simulink model "FS_PWT_Control_and_Motor"  (R2025b)
settings: Solver=FixedStepAuto  StartTime=0.0  StopTime=17  FixedStep=2e-5  RelTol=1e-3
values from neighbouring files (symbols this model uses):
  B_m = 1e-4    (= 0.0001)    [Example_parameters.m]
  Fm = 0.028    [Example_parameters.m]
  J_eq = J_m + 0.032    (= 0.032274)    [Example_parameters.m]
  Ld = 0.12e-3    (= 0.00012)    [Example_parameters.m]
  Lq = 0.24e-3    (= 0.00024)    [Example_parameters.m]
  n_max = 20000    [Example_parameters.m]
  nm_ref = n_max    (= 20000)    [Example_parameters.m]
  p = 5    [Example_parameters.m]
  R_s = 0.135    [Example_parameters.m]
  t0 = 0.2    [Example_parameters.m]
  T1 = 0.9*T_max    (= 18)    [Example_parameters.m]
  t1 = t0+5    (= 5.2)    [Example_parameters.m]
  T2 = -T_rated    (= -9.8)    [Example_parameters.m]
  t2 = t1+10    (= 15.2)    [Example_parameters.m]
  Torque_set_matrix = [379.08 379.13 379.18 379.23 379.28 379.33 379.38 379.43 379.48 379.53 379.58 379.63 ... (678 elements, 339x2)]    [Example_torque_reference.mat]
  V_dc = 600    [Example_parameters.m]
libraries: eeTransforms x3
settings Model: SimulationMode=accelerator  Creator=giuli  LastModifiedBy=giuli

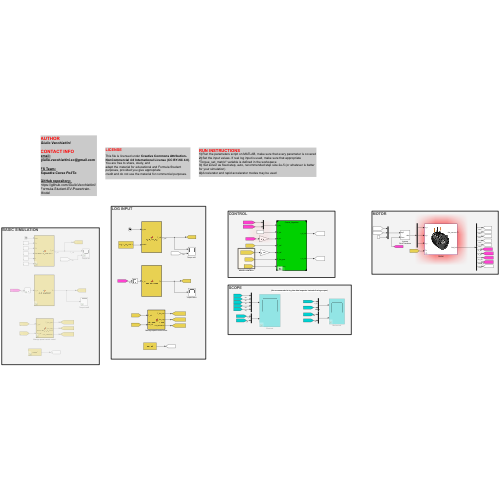
[thumbnail: Simulink's stored preview of the top-level diagram]
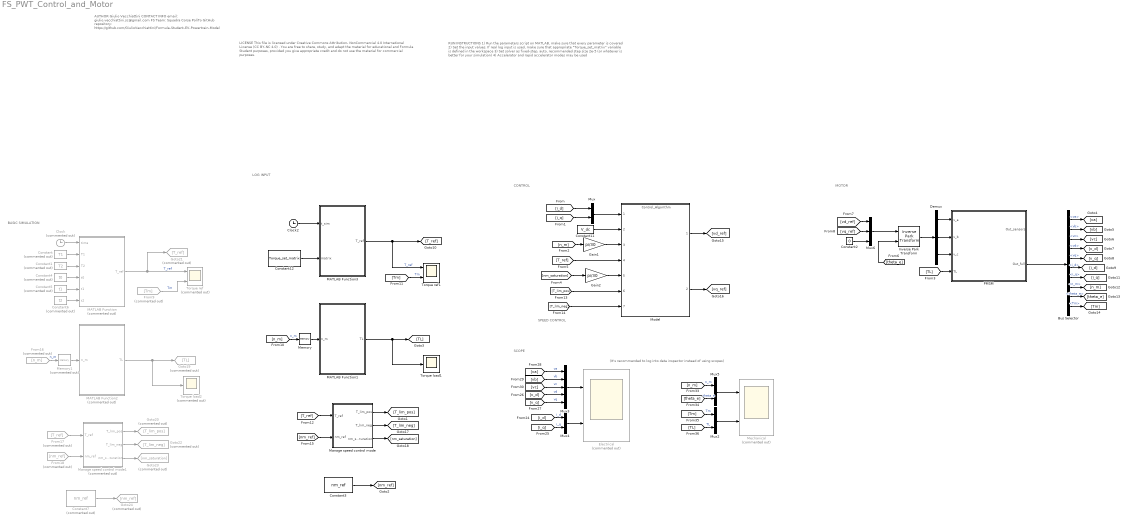
== system FS_PWT_Control_and_Motor ==
  note: (It's recommended to log into data inspector instead of using scopes)
  note: BASIC SIMULATION
  note: LOG INPUT
  note: SCOPE
  note: SPEED CONTROL
  note: CONTROL
  note: MOTOR
  note: LICENSE
      |
      | This file is licensed under Creative Commons Attribution-
      | NonCommercial 4.0 International License (CC BY-NC 4.0) . You are free to share, study, and
      | adapt the material for educational and Formula Student purposes, provided you give appropriate
      | credit and do not use the material for commercial purposes.
  note: RUN INSTRUCTIONS
      | 1) Run the parameters script on MATLAB, make sure that every parameter is covered
      | 2) Set the input values. If real log input is used, make sure that appropriate "Torque_set_matrix" variable is defined in the workspace
      | 3) Set solver as fixed-step, auto, recommended step size 2e-5 (or whatever is better for your simulation)
      | 4) Accelerator and rapid accelerator modes may be used
  note: AUTHOR
      | Giulio Vecchiattini
      |
      | CONTACT INFO
      | email: giulio.vecchiattini.sc@gmail.com
      |
      | FS Team:
      | Squadra Corse PoliTo
      |
      | GitHub repository:
      | https://github.com/GiulioVecchiattini/Formula-Student-EV-Powertrain-Model
  Bus Selector : BusSelector  OutputSignals=va,vb,vc,vd,vq,i_d,i_q,n_m,theta_e,Tm
  Clock : Clock  Commented=on
  Clock2 : Clock
  Constant : Constant  Commented=on  Value=T1
  Constant1 : Constant  Commented=on  Value=T2
  Constant11 : Constant  Value=V_dc
  Constant12 : Constant  Value=Torque_set_matrix
  Constant2 : Constant  Value=0
  Constant3 : Constant  Value=nm_ref
  Constant4 : Constant  Commented=on  Value=t0
  Constant5 : Constant  Commented=on  Value=t1
  Constant6 : Constant  Commented=on  Value=t2
  Constant7 : Constant  Commented=on  Value=nm_ref
  Demux : Demux  Outputs=3
  Electrical : Scope  Commented=on  NumInputPorts=2
      settings: ActiveDisplayYMinimum=-222.33483903014351  ActiveDisplayYMaximum=248.98362192273623
  From16 : From  Commented=on  GotoTag=n_m
  From17 : From  Commented=on  GotoTag=T_ref
  From18 : From  Commented=on  GotoTag=nm_ref
  From9 : From  Commented=on  GotoTag=Tm
  Gain1 : Gain  Gain=pi/30
  Gain2 : Gain  Gain=pi/30
  Goto19 : Goto  Commented=on  GotoTag=TL
  Goto20 : Goto  Commented=on  GotoTag=T_lim_pos
  Goto21 : Goto  Commented=on  GotoTag=T_ref
  Goto22 : Goto  Commented=on  GotoTag=T_lim_neg
  Goto23 : Goto  Commented=on  GotoTag=nm_saturation
  Goto24 : Goto  Commented=on  GotoTag=nm_ref
  Inverse Park Transform : eeTransforms/Inverse Park Transform  AxisAlignment=D-axis  PowerInvariant=off
      settings: LibrarySourceBlock=|
      | ee_sl_lib/Mathematical
      | Transforms/Inverse
      | Park Transform
  MATLAB Function : MATLAB Function  Commented=on  TreatAsAtomicUnit=on
  MATLAB Function1 : MATLAB Function  TreatAsAtomicUnit=on
  MATLAB Function2 : MATLAB Function  Commented=on  TreatAsAtomicUnit=on
  MATLAB Function3 : MATLAB Function  TreatAsAtomicUnit=on
  Manage speed control mode : MATLAB Function  TreatAsAtomicUnit=on
  Manage speed control mode1 : MATLAB Function  Commented=on  TreatAsAtomicUnit=on
  Mechanical : Scope  Commented=on  NumInputPorts=2
      settings: ActiveDisplayYMinimum=-1910.5368954552505  ActiveDisplayYMaximum=17194.832059097258  DataLoggingVariableName=ScopeData2
  Memory : Memory
  Memory1 : Memory  Commented=on
  Model : ModelReference  ModelNameDialog=Control_Algorithm.slxp  UsingDefaultArgumentValue=0,0,0,0,0,0,0,0,0,0,0,0,0,0,0,0,0,0,0  ModelReferenceVersion=1.7  CopyOfModelProtected=on  Torque_control=1  T_max=T_max  V_dc_max=V_dc_max  V_max=V_max  k_T=k_T  I_max=I_max  Kp_d=Kp_d  Ki_d=Ki_d  Kp_q=Kp_q  Ki_q=Ki_q  Kp_n=Kp_n  Ki_n=Ki_n  Kd_n=Kd_n  Kp_v=Kp_v  Ki_v=Ki_v  n_lim_brake=0.02*n_max  n_min_brake=0.01*n_max  n_max=n_max*1.02  n_lim=0.95*n_max
  Mux{,2,4..5} (4 alike) : Mux  Inputs=2
  Mux3 : Mux  Inputs=5
  Mux6 : Mux  Inputs=3
  PMSM : Subsystem  mask(PMSM){Ld=Ld, Lq=Lq, Fm=Fm, R_s=R_s, p=p, J_eq=J_eq, B_m=B_m}
      mask prompts: Ld "Ld (H)"; Lq "Lq (H)"; Fm "Magnet flux linkage (Vs)"; R_s "Rs (Ohm)"; p "Pole pairs p"; J_eq "Equivalent inertia [kg*m^2]"; B_m "Viscous friction [N*s/m]"
      mask help: Simplified PMSM with constant Ld, Lq, Fm
      mask Display: image('PMSM.jpg');
  Torque load1 : Scope
      settings: ActiveDisplayYMinimum=-1.2249999999999999  ActiveDisplayYMaximum=11.025  DataLoggingVariableName=ScopeData4
  Torque load2 : Scope  Commented=on
      settings: ActiveDisplayYMinimum=-1.2249999999999999  ActiveDisplayYMaximum=11.025
  Torque ref : Scope  Commented=on  NumInputPorts=2
      settings: ActiveDisplayYMinimum=-25.856939038681524  ActiveDisplayYMaximum=25.9527334054476  DataLoggingVariableName=ScopeData3
  Torque ref1 : Scope  NumInputPorts=2
      settings: ActiveDisplayYMinimum=-1.08125401214301  ActiveDisplayYMaximum=9.7312861092870921  DataLoggingVariableName=ScopeData5
  wires:
  Model/1 -> [vd_ref]
  Manage speed control mode/2(T_lim_neg) -> [T_lim_neg]
  [nm_saturation] -> Gain2/1
  Bus Selector/6 -> [i_d]  "<i_d>"
  Mux4/1 -> Electrical/2
  [v_q] -> Mux3/5  "vq"
  Bus Selector/3 -> [vc]  "<vc>"
  Constant5/1 -> MATLAB Function/5(t1)
  Constant11/1 -> Model/2
  [i_q] -> Mux4/2  "i_q"
  Gain2/1 -> Model/5
  Constant6/1 -> MATLAB Function/6(t2)
  MATLAB Function/1(T_ref) -> Goto21/1, Torque ref/1  "T_ref"
  Manage speed control mode/1(T_lim_pos) -> [T_lim_pos]
  From9/1 -> Torque ref/2  "Tm"
  [vd_ref] -> Mux6/1
  [vc] -> Mux3/3  "vc"
  Constant/1 -> MATLAB Function/2(T1)
  Bus Selector/9 -> [theta_e]  "<theta_e>"
  Mux2/1 -> Mechanical/2
  [T_ref] -> Manage speed control mode/1(T_ref)
  Demux/2 -> PMSM/2(v_b)
  Demux/3 -> PMSM/3(v_c)
  Constant12/1 -> MATLAB Function3/2(matrix)
  Bus Selector/10 -> [Tm]  "<Tm>"
  Bus Selector/8 -> [n_m]  "<n_m>"
  Constant3/1 -> [nm_ref]
  Mux6/1 -> Inverse Park Transform/1
  Bus Selector/5 -> [v_q]  "<vq>"
  Clock/1 -> MATLAB Function/1(time)
  [i_d] -> Mux/1
  [TL] -> Mux2/2  "TL"
  [Tm] -> Torque ref1/2  "Tm"
  Inverse Park Transform/1 -> Demux/1
  [T_ref] -> Model/4
  [va] -> Mux3/1  "va"
  MATLAB Function3/1(T_ref) -> [T_ref], Torque ref1/1  "T_ref"
  [n_m] -> Gain1/1
  Manage speed control mode/3(nm_saturation) -> [nm_saturation]
  [TL] -> PMSM/4(TL)
  [theta_e] -> Mux5/2  "theta_e"
  [n_m] -> Memory/1  "n_m"
  Memory/1 -> MATLAB Function1/1(n_m)
  Bus Selector/7 -> [i_q]  "<i_q>"
  [T_lim_neg] -> Model/7
  [Tm] -> Mux2/1  "Tm"
  Constant2/1 -> Mux6/3
  [i_d] -> Mux4/1  "i_d"
  [nm_ref] -> Manage speed control mode/2(nm_ref)
  Constant1/1 -> MATLAB Function/3(T2)
  [theta_e] -> Inverse Park Transform/2
  PMSM/2(Out_full) -> Bus Selector/1
  Constant4/1 -> MATLAB Function/4(t0)
  Bus Selector/4 -> [v_d]  "<vd>"
  Bus Selector/2 -> [vb]  "<vb>"
  Mux5/1 -> Mechanical/1
  [n_m] -> Mux5/1  "n_m"
  Mux3/1 -> Electrical/1
  Clock2/1 -> MATLAB Function3/1(t_sim)
  Mux/1 -> Model/1
  [T_lim_pos] -> Model/6
  Demux/1 -> PMSM/1(v_a)
  Model/2 -> [vq_ref]
  Bus Selector/1 -> [va]  "<va>"
  [v_d] -> Mux3/4  "vd"
  [i_q] -> Mux/2
  [vq_ref] -> Mux6/2
  Gain1/1 -> Model/3
  [vb] -> Mux3/2  "vb"
  MATLAB Function1/1(TL) -> [TL], Torque load1/1
  MATLAB Function2/1(TL) -> Goto19/1, Torque load2/1
  Memory1/1 -> MATLAB Function2/1(n_m)
  From16/1 -> Memory1/1  "n_m"
  From18/1 -> Manage speed control mode1/2(nm_ref)
  Manage speed control mode1/3(nm_saturation) -> Goto23/1
  From17/1 -> Manage speed control mode1/1(T_ref)
  Manage speed control mode1/1(T_lim_pos) -> Goto20/1
  Manage speed control mode1/2(T_lim_neg) -> Goto22/1
  Constant7/1 -> Goto24/1

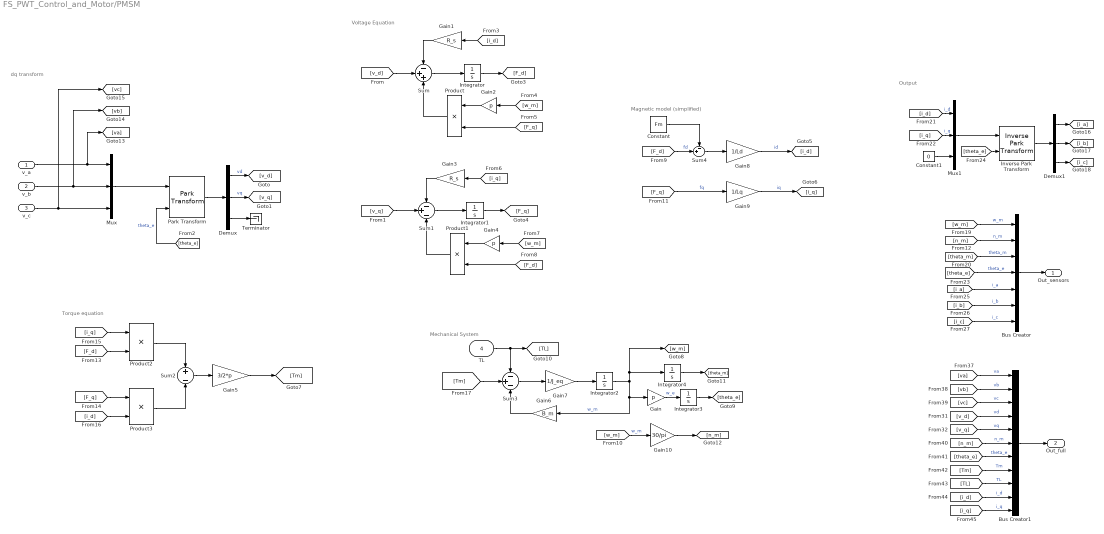
== system FS_PWT_Control_and_Motor/PMSM ==
  note: Output
  note: Magnetic model (simplified)
  note: Mechanical System
  note: Torque equation
  note: dq transform
  note: Voltage Equation
  v_a : Inport
  v_b : Inport  Port=2
  v_c : Inport  Port=3
  TL : Inport  Port=4
  Bus Creator : BusCreator  Inputs=7
  Bus Creator1 : BusCreator  Inputs=11
  Constant : Constant  Value=Fm
  Constant1 : Constant  Value=0
  Demux : Demux  Outputs=3
  Demux1 : Demux  Outputs=3
  Gain : Gain  Gain=p
  Gain1 : Gain  Gain=R_s
  Gain10 : Gain  Gain=30/pi
  Gain2 : Gain  Gain=p
  Gain3 : Gain  Gain=R_s
  Gain4 : Gain  Gain=p
  Gain5 : Gain  Gain=3/2*p
  Gain6 : Gain  Gain=B_m
  Gain7 : Gain  Gain=1/J_eq
  Gain8 : Gain  Gain=1/Ld
  Gain9 : Gain  Gain=1/Lq
  Integrator : Integrator  InitialCondition=Fm
  Integrator1 : Integrator
  Integrator2 : Integrator
  Integrator3 : Integrator  WrapState=on  WrappedStateUpperValue=2*pi  WrappedStateLowerValue=0
  Integrator4 : Integrator  WrapState=on  WrappedStateUpperValue=2*pi  WrappedStateLowerValue=0
  Inverse Park Transform : eeTransforms/Inverse Park Transform  AxisAlignment=D-axis  PowerInvariant=off
      settings: LibrarySourceBlock=|
      | ee_sl_lib/Mathematical
      | Transforms/Inverse
      | Park Transform
  Mux : Mux  Inputs=3
  Mux1 : Mux  Inputs=3
  Park Transform : eeTransforms/Park Transform  AxisAlignment=D-axis  PowerInvariant=off
      settings: LibrarySourceBlock=|
      | ee_sl_lib/Mathematical
      | Transforms/Park Transform
  Product{,1..3} (4 alike) : Product
  Sum : Sum  Inputs=-++
  Sum1 : Sum  Inputs=-+-
  Sum2 : Sum  Inputs=+|-
  Sum3 : Sum  Inputs=-+-
  Sum4 : Sum  Inputs=-+|
  Terminator : Terminator
  Out_sensors : Outport
  Out_full : Outport  Port=2
  wires:
  v_a/1 -> [va], Mux/1
  v_b/1 -> Mux/2, [vb]
  v_c/1 -> [vc], Mux/3
  Park Transform/1 -> Demux/1
  Demux/1 -> [v_d]  "vd"
  Demux/2 -> [v_q]  "vq"
  Gain1/1 -> Sum/1
  [v_d] -> Sum/2
  [i_d] -> Gain1/1
  Gain2/1 -> Product/1
  Product/1 -> Sum/3
  [w_m] -> Gain2/1
  Demux/3 -> Terminator/1
  Sum/1 -> Integrator/1
  Integrator/1 -> [F_d]
  Integrator1/1 -> [F_q]
  Sum1/1 -> Integrator1/1
  [w_m] -> Gain4/1
  Product1/1 -> Sum1/3
  Gain4/1 -> Product1/1
  [i_q] -> Gain3/1
  Gain3/1 -> Sum1/1
  [v_q] -> Sum1/2
  [F_d] -> Sum4/2  "fd"
  Gain8/1 -> [i_d]  "id"
  [F_q] -> Gain9/1  "fq"
  [i_q] -> Product2/1
  [F_d] -> Product2/2
  [F_q] -> Product3/1
  [i_d] -> Product3/2
  Product2/1 -> Sum2/1
  Product3/1 -> Sum2/2
  Sum2/1 -> Gain5/1
  Gain5/1 -> [Tm]
  TL/1 -> Sum3/1, [TL]
  [Tm] -> Sum3/2
  Gain6/1 -> Sum3/3
  Sum3/1 -> Gain7/1
  Gain7/1 -> Integrator2/1
  Integrator2/1 -> Integrator4/1, [w_m], Gain/1, Gain6/1  "w_m"
  Integrator3/1 -> [theta_e]
  [w_m] -> Bus Creator/1  "w_m"
  [theta_m] -> Bus Creator/3  "theta_m"
  Bus Creator/1 -> Out_sensors/1
  Mux/1 -> Park Transform/1
  Gain/1 -> Integrator3/1  "w_e"
  Integrator4/1 -> [theta_m]
  [theta_e] -> Bus Creator/4  "theta_e"
  [theta_e] -> Park Transform/2  "theta_e"
  [F_q] -> Product/2
  [F_d] -> Product1/2
  Constant/1 -> Sum4/1
  Sum4/1 -> Gain8/1
  Gain9/1 -> [i_q]  "iq"
  [w_m] -> Gain10/1  "w_m"
  Gain10/1 -> [n_m]
  [n_m] -> Bus Creator/2  "n_m"
  [v_q] -> Bus Creator1/5  "vq"
  [v_d] -> Bus Creator1/4  "vd"
  [vc] -> Bus Creator1/3  "vc"
  [vb] -> Bus Creator1/2  "vb"
  [va] -> Bus Creator1/1  "va"
  [n_m] -> Bus Creator1/6  "n_m"
  [theta_e] -> Bus Creator1/7  "theta_e"
  [Tm] -> Bus Creator1/8  "Tm"
  [TL] -> Bus Creator1/9  "TL"
  [i_d] -> Bus Creator1/10  "i_d"
  [i_q] -> Bus Creator1/11  "i_q"
  Bus Creator1/1 -> Out_full/1
  [i_d] -> Mux1/1  "i_d"
  [i_q] -> Mux1/2  "i_q"
  Constant1/1 -> Mux1/3
  Mux1/1 -> Inverse Park Transform/1
  [theta_e] -> Inverse Park Transform/2
  Inverse Park Transform/1 -> Demux1/1
  Demux1/1 -> [i_a]
  Demux1/2 -> [i_b]
  Demux1/3 -> [i_c]
  [i_a] -> Bus Creator/5  "i_a"
  [i_b] -> Bus Creator/6  "i_b"
  [i_c] -> Bus Creator/7  "i_c"

== matlab function FS_PWT_Control_and_Motor/MATLAB Function1 ==
  data: TL output; n_m input
function TL  = Load_simulation(n_m)

%Simplified ln_min = 300;oad modeling
%K_l, K_q, K0 set as example 

w_m = n_m*pi/30;
n_min = 300;

K_l = 1*10^(-5)*pi/30;
K_q = 2*10^(-5)*pi/30;
K0 = 1;
TL = 0;

%If speed is too low, set torque as zero 
if w_m < n_min*pi/30
    TL = 0;
else
    TL = K0 + K_l*w_m + K_q*w_m^2;

end

== matlab function FS_PWT_Control_and_Motor/MATLAB Function ==
  data: time input; T_ref output; T1 input; T2 input; t0 input; t1 input; t2 input
function T_ref  = Reference_simulation(time, T1,T2, t0, t1, t2)

T_ref = 0;

if time > 0 && time <= t0
    T_ref = 0;

elseif time > t0 && time <= t1
    T_ref = T1;

elseif time > t1 && time <= t1+0.1
    T_ref = T1+(T2-T1)/0.1*(time-t1);

elseif time > t1+0.1 && time <= t2
    T_ref = T2;

elseif time > t2
    T_ref = 0;

end

== matlab function FS_PWT_Control_and_Motor/MATLAB Function2 ==
  data: TL output; n_m input
function TL  = Load_simulation(n_m)

%Simplified ln_min = 300;oad modeling
%K_l, K_q, K0 set as example 

w_m = n_m*pi/30;
n_min = 300;

K_l = 1*10^(-5)*pi/30;
K_q = 2*10^(-5)*pi/30;
K0 = 1;
TL = 0;

%If speed is too low, set torque as zero 
if w_m < n_min*pi/30
    TL = 0;
else
    TL = K0 + K_l*w_m + K_q*w_m^2;

end

== matlab function FS_PWT_Control_and_Motor/Manage speed control mode1 ==
  data: T_lim_pos output; T_ref input; T_lim_neg output; nm_ref input; nm_saturation output
function [T_lim_pos, T_lim_neg, nm_saturation]  = Compute_T_n_limits(T_ref, nm_ref)

%Acceleration
if T_ref >= 0
    T_lim_pos = T_ref;
    T_lim_neg = 0;
    nm_saturation = nm_ref;

%Braking
else
    T_lim_pos = 0;
    T_lim_neg = T_ref;
    nm_saturation = -nm_ref;
end

== matlab function FS_PWT_Control_and_Motor/MATLAB Function3 ==
  data: t_sim input; T_ref output; matrix input
function T_ref = input_from_log(t_sim, matrix)
% Input:
%   t_sim   : current time of the Simulink simulation (scalar >= 0)
%   matrice : Nx2 matrix [time_table, torque_table]
% Output:
%   T_ref   : linearly interpolated reference torque

    % Time and torque vectors extracted from the matrix
    t_data = matrix(:, 1);
    T_data = matrix(:, 2);
    
    % Time shift: when t_sim = 0, t_target corresponds to t_data(1)
    t_target = t_sim + t_data(1);
    
    % Handling time limits (saturation at the boundaries)
    if t_target <= t_data(1)
        T_ref = T_data(1);
    elseif t_target >= t_data(end)
        T_ref = T_data(end);
    else
        % Search for the interval k such that: t_data(k) <= t_target <= t_data(k+1)
        idx = 1;
        for k = 1:length(t_data)-1
            if t_target >= t_data(k) && t_target <= t_data(k+1)
                idx = k;
                break;
            end
        end
        
        % Coordinates of the two segment endpoints
        t0 = t_data(idx);
        t1 = t_data(idx+1);
        y0 = T_data(idx);
        y1 = T_data(idx+1);
        
        % Linear interpolation formula
        dt = t1 - t0;
        if dt > 0
            alpha = (t_target - t0) / dt;
            T_ref = y0 + alpha * (y1 - y0);
        else
            T_ref = y0; % Protection against possible consecutive coincident time instances
        end
    end
end

== matlab function FS_PWT_Control_and_Motor/Manage speed control mode ==
  data: T_lim_pos output; T_ref input; T_lim_neg output; nm_ref input; nm_saturation output
function [T_lim_pos, T_lim_neg, nm_saturation]  = Compute_T_n_limits(T_ref, nm_ref)

%Acceleration
if T_ref >= 0
    T_lim_pos = T_ref;
    T_lim_neg = 0;
    nm_saturation = nm_ref;

%Braking
else
    T_lim_pos = 0;
    T_lim_neg = T_ref;
    nm_saturation = -nm_ref;
end
